simulink model "sistema_velocidad"  (R2024b)
settings: Solver=VariableStepAuto  StartTime=0.0  StopTime=tfin+ts  FixedStep=ts  MaxStep=ts  RelTol=1e-6  AbsTol=1e-9
values from neighbouring files (symbols this model uses):
  th = [0.00207452760074 0.0610946451897 0.07411845842]    [Ensayo K250 17_42.mat]    (also in ajuste_velocidad.m = thaux)
  ts = 0.02    [Ensayo K250 17_42.mat]    (also in ajuste_velocidad.m)
settings Model: Creator=zamora  LastModifiedBy=ramonimac
settings SolverCC: AutoScaleAbsTol=off  ZeroCrossAlgorithm=Adaptive  AlgebraicLoopSolver=TrustRegion
settings DataIOCC: SaveFormat=Array  SignalLoggingSaveFormat=ModelDataLogs  SaveOutput=off  SaveTime=off  ReturnWorkspaceOutputs=off  StateSaveName=x  TimeSaveName=t  OutputSaveName=y
settings OptimizationCC: BlockReduction=off  BooleanDataType=off  DefaultParameterBehavior=Inlined  BufferReuse=off  ExpressionDepthLimit=2147483647  LifeSpan=inf
settings DebuggingCC: SaveWithParameterizedLinksMsg=none  UnderspecifiedInitializationDetection=Classic  MergeDetectMultiDrivingBlocksExec=none  SignalResolutionControl=TryResolveAllWithWarning  MaxConsecutiveZCsMsg=none  IgnoredZcDiagnostic=none  MultiTaskDSMMsg=warning  MultiTaskCondExecSysMsg=none  FcnCallInpInsideContextMsg=warning  UnconnectedInputMsg=warning  UnconnectedOutputMsg=warning  UnconnectedLineMsg=warning  StateNameClashWarn=warning  SFUnexpectedBacktrackingDiag=warning  SFNoUnconditionalDefaultTransitionDiag=warning  SFExecutionAtInitializationDiag=none  ArithmeticOperatorsInVariantConditions=warning
settings HardwareCC: ProdBitPerPointer=32  ProdBitPerSizeT=32  ProdBitPerPtrDiffT=32  ProdLargestAtomicFloat=None  ProdIntDivRoundTo=Undefined  ProdEndianess=Unspecified  ProdWordSize=32  ProdHWDeviceType=32-bit Generic  TargetUnknown=on
settings ModelReferenceCC: EnableRefExpFcnMdlSchedulingChecks=on  PropagateSignalLabelsOutOfModel=off
settings SFSimCC: SimUseLocalCustomCode=off  CustomCodeUndefinedFunction=UseInterfaceOnly
settings RTWCC: TemplateMakefile=grt_unix.tmf  RTWUseLocalCustomCode=off  GPUComputeCapability=3.5
settings CodeAppCC: StateflowObjectComments=on
settings GRTTargetCC: TargetLangStandard=C89/C90 (ANSI)  CombineOutputUpdateFcns=off  GRTInterface=on
settings ConfigComp: CovMetricSettings=dw  CovSaveCumulativeToWorkspaceVar=on  CovSaveSingleToWorkspaceVar=on  CovExternalEMLEnable=off  CovSFcnEnable=off

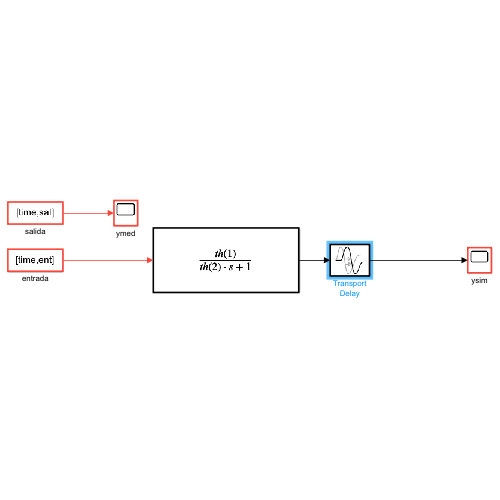
[thumbnail: Simulink's stored preview of the top-level diagram]
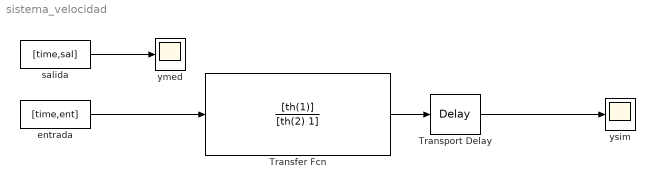
== system sistema_velocidad ==
  Transfer Fcn : TransferFcn  Numerator=[th(1)]  Denominator=[th(2) 1]
  Transport Delay : TransportDelay  DelayTime=th(3)
  entrada : FromWorkspace  VariableName=[time,ent]  SampleTime=ts
  salida : FromWorkspace  VariableName=[time,sal]  SampleTime=ts
  ymed : Scope
  ysim : Scope
  wires:
  salida/1 -> ymed/1
  Transport Delay/1 -> ysim/1
  Transfer Fcn/1 -> Transport Delay/1
  entrada/1 -> Transfer Fcn/1
